simulink model "drive_cmd_pack"  (R2026b)
settings: Solver=VariableStepAuto
undefined symbols (not defined in the file or in its folder): P
libraries: simulink x2, svdutilitieslib x1
settings Model: Creator=aomar  LastModifiedBy=aomar

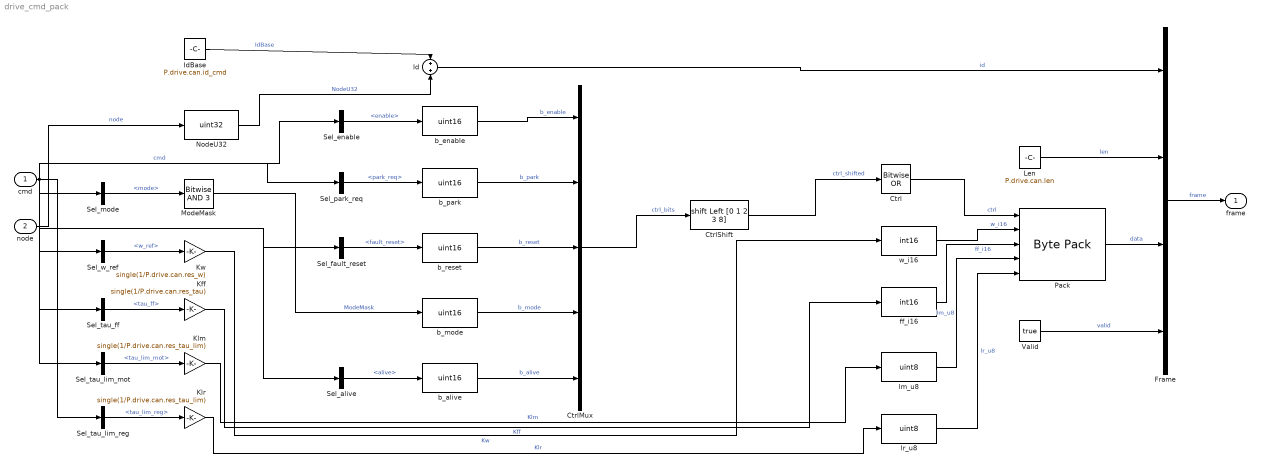
== system drive_cmd_pack ==
  cmd : Inport  OutDataTypeStr=Bus: Bus_DriveSideCmd
  node : Inport  Port=2  OutDataTypeStr=uint8
  Ctrl : simulink/Logic and Bit Operations/Bitwise Operator  logicop=OR  UseBitMask=off  BitMask=bin2dec('11011001')  BitMaskRealWorld=Stored Integer
  CtrlMux : Mux  Inputs=5
  CtrlShift : ArithShift  BitShiftNumber=[0 1 2 3 8]  BitShiftDirection=Left
  Frame : BusCreator  Inputs=4  OutDataTypeStr=Bus: Bus_CanFrame8  NonVirtualBus=on
  Id : Sum  OutDataTypeStr=uint32  SaturateOnIntegerOverflow=on
  IdBase : Constant  Value=P.drive.can.id_cmd  OutDataTypeStr=uint32
  Kff : Gain  Gain=single(1/P.drive.can.res_tau)
  Klm : Gain  Gain=single(1/P.drive.can.res_tau_lim)
  Klr : Gain  Gain=single(1/P.drive.can.res_tau_lim)
  Kw : Gain  Gain=single(1/P.drive.can.res_w)
  Len : Constant  Value=P.drive.can.len  OutDataTypeStr=uint8
  ModeMask : simulink/Logic and Bit Operations/Bitwise Operator  logicop=AND  UseBitMask=on  BitMask=3  BitMaskRealWorld=Stored Integer
  NodeU32 : DataTypeConversion  OutDataTypeStr=uint32  RndMeth=Nearest
  Pack : svdutilitieslib/Byte Pack  maskPackedDataType=uint8  datatypes={'uint16','int16','int16','uint8','uint8'}  byteAlign=1  blockPlatform=arduinoert
      settings: LibrarySourceBlock=mcblib/Signal Management/Byte Pack
  Sel_alive : BusSelector  OutputSignals=alive
  Sel_enable : BusSelector  OutputSignals=enable
  Sel_fault_reset : BusSelector  OutputSignals=fault_reset
  Sel_mode : BusSelector  OutputSignals=mode
  Sel_park_req : BusSelector  OutputSignals=park_req
  Sel_tau_ff : BusSelector  OutputSignals=tau_ff
  Sel_tau_lim_mot : BusSelector  OutputSignals=tau_lim_mot
  Sel_tau_lim_reg : BusSelector  OutputSignals=tau_lim_reg
  Sel_w_ref : BusSelector  OutputSignals=w_ref
  Valid : Constant  Value=true  OutDataTypeStr=boolean
  b_alive : DataTypeConversion  OutDataTypeStr=uint16  RndMeth=Nearest
  b_enable : DataTypeConversion  OutDataTypeStr=uint16  RndMeth=Nearest
  b_mode : DataTypeConversion  OutDataTypeStr=uint16  RndMeth=Nearest
  b_park : DataTypeConversion  OutDataTypeStr=uint16  RndMeth=Nearest
  b_reset : DataTypeConversion  OutDataTypeStr=uint16  RndMeth=Nearest
  ff_i16 : DataTypeConversion  OutDataTypeStr=int16  RndMeth=Nearest
  lm_u8 : DataTypeConversion  OutDataTypeStr=uint8  RndMeth=Nearest
  lr_u8 : DataTypeConversion  OutDataTypeStr=uint8  RndMeth=Nearest
  w_i16 : DataTypeConversion  OutDataTypeStr=int16  RndMeth=Nearest
  frame : Outport  OutDataTypeStr=Bus: Bus_CanFrame8
  wires:
  cmd/1 -> Sel_tau_lim_reg/1, Sel_alive/1, Sel_tau_lim_mot/1, Sel_tau_ff/1, Sel_w_ref/1, Sel_fault_reset/1, Sel_enable/1, Sel_mode/1, Sel_park_req/1  "cmd"
  node/1 -> NodeU32/1  "node"
  Sel_mode/1 -> ModeMask/1  "<mode>"
  Sel_w_ref/1 -> Kw/1  "<w_ref>"
  Sel_tau_ff/1 -> Kff/1  "<tau_ff>"
  Sel_tau_lim_mot/1 -> Klm/1  "<tau_lim_mot>"
  Sel_tau_lim_reg/1 -> Klr/1  "<tau_lim_reg>"
  IdBase/1 -> Id/1  "IdBase"
  Kw/1 -> w_i16/1  "Kw"
  Kff/1 -> ff_i16/1  "Kff"
  Klm/1 -> lm_u8/1  "Klm"
  Klr/1 -> lr_u8/1  "Klr"
  ModeMask/1 -> b_mode/1  "ModeMask"
  NodeU32/1 -> Id/2  "NodeU32"
  Sel_enable/1 -> b_enable/1  "<enable>"
  Sel_park_req/1 -> b_park/1  "<park_req>"
  Sel_fault_reset/1 -> b_reset/1  "<fault_reset>"
  Sel_alive/1 -> b_alive/1  "<alive>"
  Id/1 -> Frame/1  "id"
  b_enable/1 -> CtrlMux/1  "b_enable"
  b_park/1 -> CtrlMux/2  "b_park"
  b_reset/1 -> CtrlMux/3  "b_reset"
  b_mode/1 -> CtrlMux/4  "b_mode"
  b_alive/1 -> CtrlMux/5  "b_alive"
  CtrlMux/1 -> CtrlShift/1  "ctrl_bits"
  CtrlShift/1 -> Ctrl/1  "ctrl_shifted"
  Ctrl/1 -> Pack/1  "ctrl"
  w_i16/1 -> Pack/2  "w_i16"
  ff_i16/1 -> Pack/3  "ff_i16"
  lm_u8/1 -> Pack/4  "lm_u8"
  lr_u8/1 -> Pack/5  "lr_u8"
  Len/1 -> Frame/2  "len"
  Valid/1 -> Frame/4  "valid"
  Pack/1 -> Frame/3  "data"
  Frame/1 -> frame/1  "frame"
